simulink model "substation_132_13_8kv_digital_twin"  (R2023b)
settings: Solver=ode23tb  StartTime=0.0  StopTime=1.0  MaxStep=100e-6  RelTol=1e-3
settings Model: Creator=ASUS  LastModifiedBy=ASUS

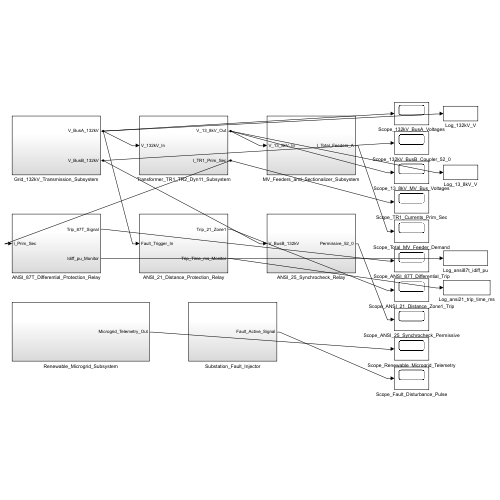
[thumbnail: Simulink's stored preview of the top-level diagram]
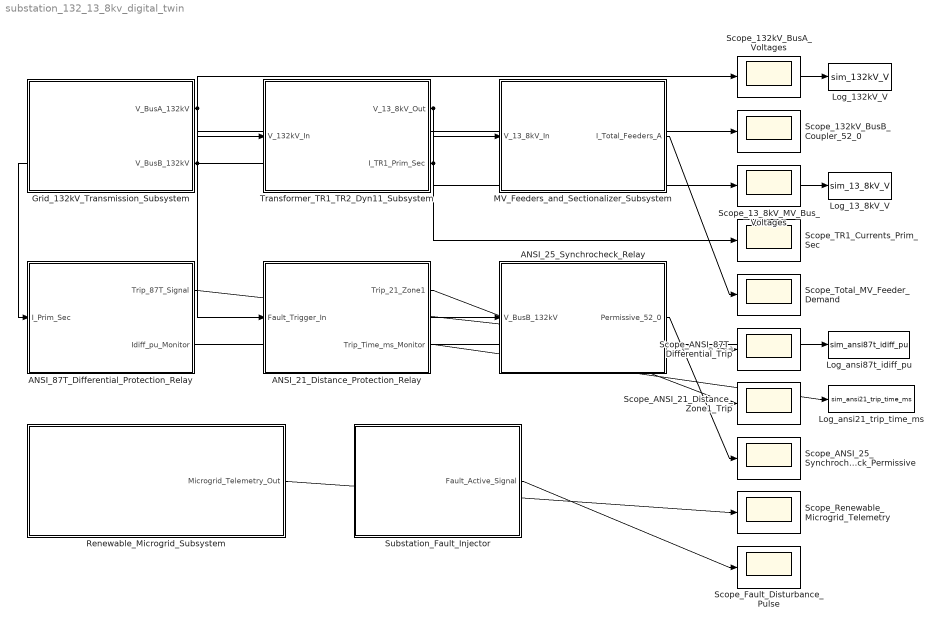
== system substation_132_13_8kv_digital_twin ==
  ANSI_21_Distance_Protection_Relay : Subsystem
  ANSI_25_Synchrocheck_Relay : Subsystem
  ANSI_87T_Differential_Protection_Relay : Subsystem
  Grid_132kV_Transmission_Subsystem : Subsystem
  Log_132kV_V : ToWorkspace  VariableName=sim_132kV_V  SampleTime=-1
  Log_13_8kV_V : ToWorkspace  VariableName=sim_13_8kV_V  SampleTime=-1
  Log_ansi21_trip_time_ms : ToWorkspace  VariableName=sim_ansi21_trip_time_ms  SampleTime=-1
  Log_ansi87t_idiff_pu : ToWorkspace  VariableName=sim_ansi87t_idiff_pu  SampleTime=-1
  MV_Feeders_and_Sectionalizer_Subsystem : Subsystem
  Renewable_Microgrid_Subsystem : Subsystem
  Scope_132kV_BusA_Voltages : Scope
  Scope_132kV_BusB_Coupler_52_0 : Scope
  Scope_13_8kV_MV_Bus_Voltages : Scope
  Scope_ANSI_21_Distance_Zone1_Trip : Scope
  Scope_ANSI_25_Synchrocheck_Permissive : Scope
  Scope_ANSI_87T_Differential_Trip : Scope
  Scope_Fault_Disturbance_Pulse : Scope
  Scope_Renewable_Microgrid_Telemetry : Scope
  Scope_TR1_Currents_Prim_Sec : Scope
  Scope_Total_MV_Feeder_Demand : Scope
  Substation_Fault_Injector : Subsystem
  Transformer_TR1_TR2_Dyn11_Subsystem : Subsystem
  wires:
  Grid_132kV_Transmission_Subsystem/1(V_BusA_132kV) -> Scope_132kV_BusA_Voltages/1, Log_132kV_V/1, Transformer_TR1_TR2_Dyn11_Subsystem/1(V_132kV_In), ANSI_21_Distance_Protection_Relay/1(Fault_Trigger_In)
  Grid_132kV_Transmission_Subsystem/2(V_BusB_132kV) -> Scope_132kV_BusB_Coupler_52_0/1, ANSI_25_Synchrocheck_Relay/1(V_BusB_132kV)
  Transformer_TR1_TR2_Dyn11_Subsystem/1(V_13_8kV_Out) -> Scope_13_8kV_MV_Bus_Voltages/1, Log_13_8kV_V/1, MV_Feeders_and_Sectionalizer_Subsystem/1(V_13_8kV_In)
  Transformer_TR1_TR2_Dyn11_Subsystem/2(I_TR1_Prim_Sec) -> Scope_TR1_Currents_Prim_Sec/1, ANSI_87T_Differential_Protection_Relay/1(I_Prim_Sec)
  MV_Feeders_and_Sectionalizer_Subsystem/1(I_Total_Feeders_A) -> Scope_Total_MV_Feeder_Demand/1
  ANSI_87T_Differential_Protection_Relay/1(Trip_87T_Signal) -> Scope_ANSI_87T_Differential_Trip/1
  ANSI_87T_Differential_Protection_Relay/2(Idiff_pu_Monitor) -> Log_ansi87t_idiff_pu/1
  ANSI_21_Distance_Protection_Relay/2(Trip_Time_ms_Monitor) -> Log_ansi21_trip_time_ms/1
  ANSI_21_Distance_Protection_Relay/1(Trip_21_Zone1) -> Scope_ANSI_21_Distance_Zone1_Trip/1
  ANSI_25_Synchrocheck_Relay/1(Permissive_52_0) -> Scope_ANSI_25_Synchrocheck_Permissive/1
  Renewable_Microgrid_Subsystem/1(Microgrid_Telemetry_Out) -> Scope_Renewable_Microgrid_Telemetry/1
  Substation_Fault_Injector/1(Fault_Active_Signal) -> Scope_Fault_Disturbance_Pulse/1

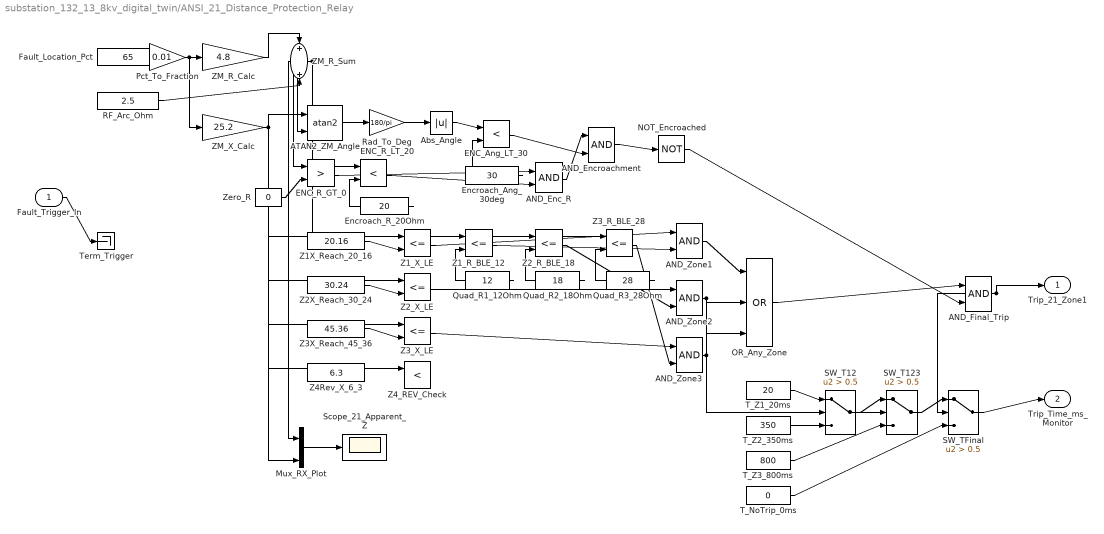
== system substation_132_13_8kv_digital_twin/ANSI_21_Distance_Protection_Relay ==
  Fault_Trigger_In : Inport
  AND_Enc_R : Logic  AllPortsSameDT=off  OutDataTypeStr=boolean
  AND_Encroachment : Logic  AllPortsSameDT=off  OutDataTypeStr=boolean
  AND_Final_Trip : Logic  AllPortsSameDT=off  OutDataTypeStr=boolean
  AND_Zone1 : Logic  AllPortsSameDT=off  OutDataTypeStr=boolean
  AND_Zone2 : Logic  AllPortsSameDT=off  OutDataTypeStr=boolean
  AND_Zone3 : Logic  AllPortsSameDT=off  OutDataTypeStr=boolean
  ATAN2_ZM_Angle : Trigonometry  Operator=atan2
  Abs_Angle : Abs  SaturateOnIntegerOverflow=off
  ENC_Ang_LT_30 : RelationalOperator  Operator=<  OutDataTypeStr=boolean  RndMeth=Simplest  InputSameDT=off
  ENC_R_GT_0 : RelationalOperator  Operator=>  OutDataTypeStr=boolean  RndMeth=Simplest  InputSameDT=off
  ENC_R_LT_20 : RelationalOperator  Operator=<  OutDataTypeStr=boolean  RndMeth=Simplest  InputSameDT=off
  Encroach_Ang_30deg : Constant  Value=30
  Encroach_R_20Ohm : Constant  Value=20
  Fault_Location_Pct : Constant  Value=65
  Mux_RX_Plot : Mux  Inputs=2
  NOT_Encroached : Logic  Operator=NOT  AllPortsSameDT=off  OutDataTypeStr=boolean
  OR_Any_Zone : Logic  Operator=OR  Inputs=3  AllPortsSameDT=off  OutDataTypeStr=boolean
  Pct_To_Fraction : Gain  Gain=0.01
  Quad_R1_12Ohm : Constant  Value=12
  Quad_R2_18Ohm : Constant  Value=18
  Quad_R3_28Ohm : Constant  Value=28
  RF_Arc_Ohm : Constant  Value=2.5
  Rad_To_Deg : Gain  Gain=180/pi
  SW_T12 : Switch  Criteria=u2 > Threshold  Threshold=0.5  SaturateOnIntegerOverflow=off  InputSameDT=off
  SW_T123 : Switch  Criteria=u2 > Threshold  Threshold=0.5  SaturateOnIntegerOverflow=off  InputSameDT=off
  SW_TFinal : Switch  Criteria=u2 > Threshold  Threshold=0.5  SaturateOnIntegerOverflow=off  InputSameDT=off
  Scope_21_Apparent_Z : Scope
  T_NoTrip_0ms : Constant  Value=0
  T_Z1_20ms : Constant  Value=20
  T_Z2_350ms : Constant  Value=350
  T_Z3_800ms : Constant  Value=800
  Term_Trigger : Terminator
  Z1X_Reach_20_16 : Constant  Value=20.16
  Z1_R_BLE_12 : RelationalOperator  Operator=<=  OutDataTypeStr=boolean  RndMeth=Simplest  InputSameDT=off
  Z1_X_LE : RelationalOperator  Operator=<=  OutDataTypeStr=boolean  RndMeth=Simplest  InputSameDT=off
  Z2X_Reach_30_24 : Constant  Value=30.24
  Z2_R_BLE_18 : RelationalOperator  Operator=<=  OutDataTypeStr=boolean  RndMeth=Simplest  InputSameDT=off
  Z2_X_LE : RelationalOperator  Operator=<=  OutDataTypeStr=boolean  RndMeth=Simplest  InputSameDT=off
  Z3X_Reach_45_36 : Constant  Value=45.36
  Z3_R_BLE_28 : RelationalOperator  Operator=<=  OutDataTypeStr=boolean  RndMeth=Simplest  InputSameDT=off
  Z3_X_LE : RelationalOperator  Operator=<=  OutDataTypeStr=boolean  RndMeth=Simplest  InputSameDT=off
  Z4Rev_X_6_3 : Constant  Value=6.3
  Z4_REV_Check : RelationalOperator  Operator=<  OutDataTypeStr=boolean  RndMeth=Simplest  InputSameDT=off
  ZM_R_Calc : Gain  Gain=4.8
  ZM_R_Sum : Sum
  ZM_X_Calc : Gain  Gain=25.2
  Zero_R : Constant  Value=0
  Trip_21_Zone1 : Outport
  Trip_Time_ms_Monitor : Outport  Port=2
  wires:
  Fault_Trigger_In/1 -> Term_Trigger/1
  Fault_Location_Pct/1 -> Pct_To_Fraction/1
  Pct_To_Fraction/1 -> ZM_R_Calc/1, ZM_X_Calc/1
  ZM_R_Calc/1 -> ZM_R_Sum/1
  RF_Arc_Ohm/1 -> ZM_R_Sum/2
  ZM_X_Calc/1 -> ATAN2_ZM_Angle/1, Z1_X_LE/1, Z2_X_LE/1, Z3_X_LE/1, Z4_REV_Check/1, Mux_RX_Plot/2
  ZM_R_Sum/1 -> ATAN2_ZM_Angle/2, ENC_R_GT_0/1, ENC_R_LT_20/1, Z1_R_BLE_12/1, Z2_R_BLE_18/1, Z3_R_BLE_28/1, Mux_RX_Plot/1
  ATAN2_ZM_Angle/1 -> Rad_To_Deg/1
  Rad_To_Deg/1 -> Abs_Angle/1
  Zero_R/1 -> ENC_R_GT_0/2
  Encroach_R_20Ohm/1 -> ENC_R_LT_20/2
  Abs_Angle/1 -> ENC_Ang_LT_30/1
  Encroach_Ang_30deg/1 -> ENC_Ang_LT_30/2
  ENC_R_GT_0/1 -> AND_Enc_R/1
  ENC_R_LT_20/1 -> AND_Enc_R/2
  AND_Enc_R/1 -> AND_Encroachment/1
  ENC_Ang_LT_30/1 -> AND_Encroachment/2
  Z1X_Reach_20_16/1 -> Z1_X_LE/2
  Z2X_Reach_30_24/1 -> Z2_X_LE/2
  Z3X_Reach_45_36/1 -> Z3_X_LE/2
  Quad_R1_12Ohm/1 -> Z1_R_BLE_12/2
  Quad_R2_18Ohm/1 -> Z2_R_BLE_18/2
  Quad_R3_28Ohm/1 -> Z3_R_BLE_28/2
  Z1_X_LE/1 -> AND_Zone1/1
  Z1_R_BLE_12/1 -> AND_Zone1/2
  Z2_X_LE/1 -> AND_Zone2/1
  Z2_R_BLE_18/1 -> AND_Zone2/2
  Z3_X_LE/1 -> AND_Zone3/1
  Z3_R_BLE_28/1 -> AND_Zone3/2
  AND_Zone1/1 -> OR_Any_Zone/1
  AND_Zone2/1 -> OR_Any_Zone/2, SW_T12/2
  AND_Zone3/1 -> OR_Any_Zone/3, SW_T123/2
  T_Z1_20ms/1 -> SW_T12/1
  T_Z2_350ms/1 -> SW_T12/3
  SW_T12/1 -> SW_T123/1
  T_Z3_800ms/1 -> SW_T123/3
  SW_T123/1 -> SW_TFinal/1
  AND_Final_Trip/1 -> SW_TFinal/2, Trip_21_Zone1/1
  T_NoTrip_0ms/1 -> SW_TFinal/3
  AND_Encroachment/1 -> NOT_Encroached/1
  OR_Any_Zone/1 -> AND_Final_Trip/1
  NOT_Encroached/1 -> AND_Final_Trip/2
  SW_TFinal/1 -> Trip_Time_ms_Monitor/1
  Mux_RX_Plot/1 -> Scope_21_Apparent_Z/1

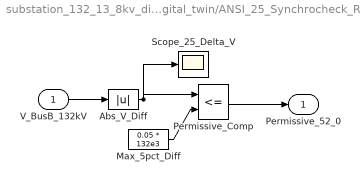
== system substation_132_13_8kv_digital_twin/ANSI_25_Synchrocheck_Relay ==
  V_BusB_132kV : Inport
  Abs_V_Diff : Abs  SaturateOnIntegerOverflow=off
  Max_5pct_Diff : Constant  Value=0.05 * 132e3
  Permissive_Comp : RelationalOperator  Operator=<=  OutDataTypeStr=boolean  RndMeth=Simplest  InputSameDT=off
  Scope_25_Delta_V : Scope
  Permissive_52_0 : Outport
  wires:
  Abs_V_Diff/1 -> Scope_25_Delta_V/1, Permissive_Comp/1
  V_BusB_132kV/1 -> Abs_V_Diff/1
  Max_5pct_Diff/1 -> Permissive_Comp/2
  Permissive_Comp/1 -> Permissive_52_0/1

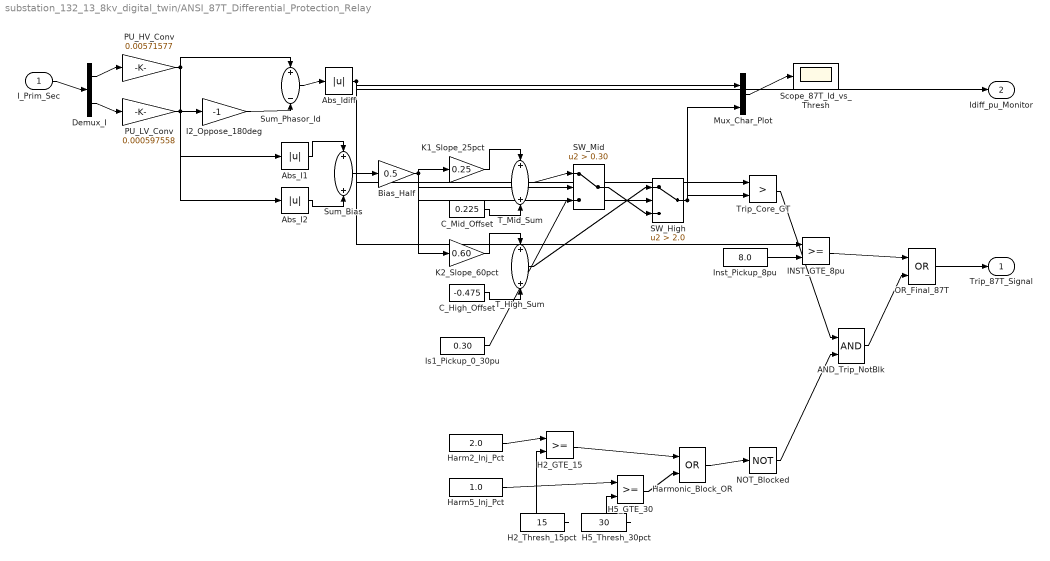
== system substation_132_13_8kv_digital_twin/ANSI_87T_Differential_Protection_Relay ==
  I_Prim_Sec : Inport
  AND_Trip_NotBlk : Logic  AllPortsSameDT=off  OutDataTypeStr=boolean
  Abs_I1 : Abs  SaturateOnIntegerOverflow=off
  Abs_I2 : Abs  SaturateOnIntegerOverflow=off
  Abs_Idiff : Abs  SaturateOnIntegerOverflow=off
  Bias_Half : Gain  Gain=0.5
  C_High_Offset : Constant  Value=-0.475
  C_Mid_Offset : Constant  Value=0.225
  Demux_I : Demux  Outputs=2
  H2_GTE_15 : RelationalOperator  OutDataTypeStr=boolean  RndMeth=Simplest  InputSameDT=off
  H2_Thresh_15pct : Constant  Value=15
  H5_GTE_30 : RelationalOperator  OutDataTypeStr=boolean  RndMeth=Simplest  InputSameDT=off
  H5_Thresh_30pct : Constant  Value=30
  Harm2_Inj_Pct : Constant  Value=2.0
  Harm5_Inj_Pct : Constant  Value=1.0
  Harmonic_Block_OR : Logic  Operator=OR  AllPortsSameDT=off  OutDataTypeStr=boolean
  I2_Oppose_180deg : Gain  Gain=-1
  INST_GTE_8pu : RelationalOperator  OutDataTypeStr=boolean  RndMeth=Simplest  InputSameDT=off
  Inst_Pickup_8pu : Constant  Value=8.0
  Is1_Pickup_0_30pu : Constant  Value=0.30
  K1_Slope_25pct : Gain  Gain=0.25
  K2_Slope_60pct : Gain  Gain=0.60
  Mux_Char_Plot : Mux  Inputs=2
  NOT_Blocked : Logic  Operator=NOT  AllPortsSameDT=off  OutDataTypeStr=boolean
  OR_Final_87T : Logic  Operator=OR  AllPortsSameDT=off  OutDataTypeStr=boolean
  PU_HV_Conv : Gain  Gain=0.00571577
  PU_LV_Conv : Gain  Gain=0.000597558
  SW_High : Switch  Criteria=u2 > Threshold  Threshold=2.0  SaturateOnIntegerOverflow=off  InputSameDT=off
  SW_Mid : Switch  Criteria=u2 > Threshold  Threshold=0.30  SaturateOnIntegerOverflow=off  InputSameDT=off
  Scope_87T_Id_vs_Thresh : Scope
  Sum_Bias : Sum
  Sum_Phasor_Id : Sum  Inputs=+-
  T_High_Sum : Sum
  T_Mid_Sum : Sum
  Trip_Core_GT : RelationalOperator  Operator=>  OutDataTypeStr=boolean  RndMeth=Simplest  InputSameDT=off
  Trip_87T_Signal : Outport
  Idiff_pu_Monitor : Outport  Port=2
  wires:
  I_Prim_Sec/1 -> Demux_I/1
  Demux_I/1 -> PU_HV_Conv/1
  Demux_I/2 -> PU_LV_Conv/1
  PU_LV_Conv/1 -> I2_Oppose_180deg/1, Abs_I2/1
  PU_HV_Conv/1 -> Sum_Phasor_Id/1, Abs_I1/1
  I2_Oppose_180deg/1 -> Sum_Phasor_Id/2
  Sum_Phasor_Id/1 -> Abs_Idiff/1
  Abs_I1/1 -> Sum_Bias/1
  Abs_I2/1 -> Sum_Bias/2
  Sum_Bias/1 -> Bias_Half/1
  Bias_Half/1 -> K1_Slope_25pct/1, K2_Slope_60pct/1, SW_Mid/2, SW_High/2
  K1_Slope_25pct/1 -> T_Mid_Sum/1
  C_Mid_Offset/1 -> T_Mid_Sum/2
  K2_Slope_60pct/1 -> T_High_Sum/1
  C_High_Offset/1 -> T_High_Sum/2
  T_Mid_Sum/1 -> SW_Mid/1
  Is1_Pickup_0_30pu/1 -> SW_Mid/3
  T_High_Sum/1 -> SW_High/1
  SW_Mid/1 -> SW_High/3
  Harm2_Inj_Pct/1 -> H2_GTE_15/1
  H2_Thresh_15pct/1 -> H2_GTE_15/2
  Harm5_Inj_Pct/1 -> H5_GTE_30/1
  H5_Thresh_30pct/1 -> H5_GTE_30/2
  H2_GTE_15/1 -> Harmonic_Block_OR/1
  H5_GTE_30/1 -> Harmonic_Block_OR/2
  Abs_Idiff/1 -> Trip_Core_GT/1, INST_GTE_8pu/1, Mux_Char_Plot/1, Idiff_pu_Monitor/1
  SW_High/1 -> Trip_Core_GT/2, Mux_Char_Plot/2
  Inst_Pickup_8pu/1 -> INST_GTE_8pu/2
  Harmonic_Block_OR/1 -> NOT_Blocked/1
  Trip_Core_GT/1 -> AND_Trip_NotBlk/1
  NOT_Blocked/1 -> AND_Trip_NotBlk/2
  INST_GTE_8pu/1 -> OR_Final_87T/1
  AND_Trip_NotBlk/1 -> OR_Final_87T/2
  OR_Final_87T/1 -> Trip_87T_Signal/1
  Mux_Char_Plot/1 -> Scope_87T_Id_vs_Thresh/1

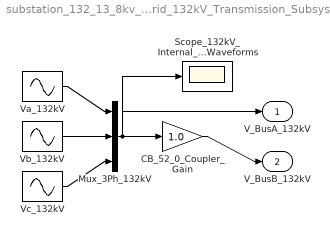
== system substation_132_13_8kv_digital_twin/Grid_132kV_Transmission_Subsystem ==
  CB_52_0_Coupler_Gain : Gain  Gain=1.0
  Mux_3Ph_132kV : Mux  Inputs=3
  Scope_132kV_Internal_Waveforms : Scope
  Va_132kV : Sin  Amplitude=132e3 * sqrt(2)/sqrt(3)  Frequency=2*pi*60  SampleTime=0
  Vb_132kV : Sin  Amplitude=132e3 * sqrt(2)/sqrt(3)  Frequency=2*pi*60  Phase=-2*pi/3  SampleTime=0
  Vc_132kV : Sin  Amplitude=132e3 * sqrt(2)/sqrt(3)  Frequency=2*pi*60  Phase=2*pi/3  SampleTime=0
  V_BusA_132kV : Outport
  V_BusB_132kV : Outport  Port=2
  wires:
  Mux_3Ph_132kV/1 -> Scope_132kV_Internal_Waveforms/1, V_BusA_132kV/1, CB_52_0_Coupler_Gain/1
  Va_132kV/1 -> Mux_3Ph_132kV/1
  Vb_132kV/1 -> Mux_3Ph_132kV/2
  Vc_132kV/1 -> Mux_3Ph_132kV/3
  CB_52_0_Coupler_Gain/1 -> V_BusB_132kV/1

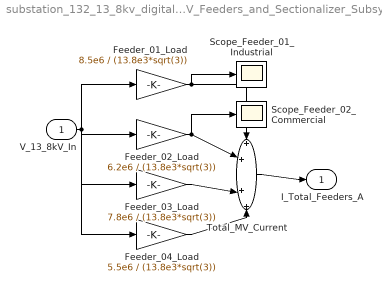
== system substation_132_13_8kv_digital_twin/MV_Feeders_and_Sectionalizer_Subsystem ==
  V_13_8kV_In : Inport
  Feeder_01_Load : Gain  Gain=8.5e6 / (13.8e3*sqrt(3))
  Feeder_02_Load : Gain  Gain=6.2e6 / (13.8e3*sqrt(3))
  Feeder_03_Load : Gain  Gain=7.8e6 / (13.8e3*sqrt(3))
  Feeder_04_Load : Gain  Gain=5.5e6 / (13.8e3*sqrt(3))
  Scope_Feeder_01_Industrial : Scope
  Scope_Feeder_02_Commercial : Scope
  Total_MV_Current : Sum  Inputs=++++
  I_Total_Feeders_A : Outport
  wires:
  Feeder_01_Load/1 -> Scope_Feeder_01_Industrial/1, Total_MV_Current/1
  Feeder_02_Load/1 -> Scope_Feeder_02_Commercial/1, Total_MV_Current/2
  V_13_8kV_In/1 -> Feeder_01_Load/1, Feeder_02_Load/1, Feeder_03_Load/1, Feeder_04_Load/1
  Feeder_03_Load/1 -> Total_MV_Current/3
  Feeder_04_Load/1 -> Total_MV_Current/4
  Total_MV_Current/1 -> I_Total_Feeders_A/1

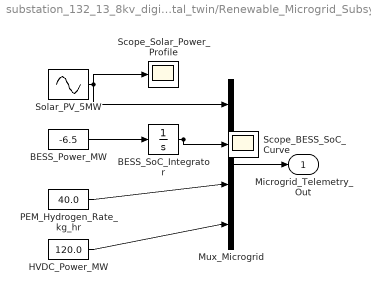
== system substation_132_13_8kv_digital_twin/Renewable_Microgrid_Subsystem ==
  BESS_Power_MW : Constant  Value=-6.5
  BESS_SoC_Integrator : Integrator  InitialCondition=72.0
  HVDC_Power_MW : Constant  Value=120.0
  Mux_Microgrid : Mux
  PEM_Hydrogen_Rate_kg_hr : Constant  Value=40.0
  Scope_BESS_SoC_Curve : Scope
  Scope_Solar_Power_Profile : Scope
  Solar_PV_5MW : Sin  Amplitude=5.0  Frequency=2*pi/24  Phase=-pi/2  SampleTime=0
  Microgrid_Telemetry_Out : Outport
  wires:
  Solar_PV_5MW/1 -> Scope_Solar_Power_Profile/1, Mux_Microgrid/1
  BESS_SoC_Integrator/1 -> Scope_BESS_SoC_Curve/1, Mux_Microgrid/2
  BESS_Power_MW/1 -> BESS_SoC_Integrator/1
  PEM_Hydrogen_Rate_kg_hr/1 -> Mux_Microgrid/3
  HVDC_Power_MW/1 -> Mux_Microgrid/4
  Mux_Microgrid/1 -> Microgrid_Telemetry_Out/1

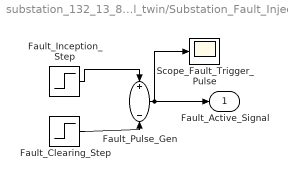
== system substation_132_13_8kv_digital_twin/Substation_Fault_Injector ==
  Fault_Clearing_Step : Step  Time=0.28  SampleTime=0
  Fault_Inception_Step : Step  Time=0.20  SampleTime=0
  Fault_Pulse_Gen : Sum  Inputs=+-
  Scope_Fault_Trigger_Pulse : Scope
  Fault_Active_Signal : Outport
  wires:
  Fault_Pulse_Gen/1 -> Scope_Fault_Trigger_Pulse/1, Fault_Active_Signal/1
  Fault_Inception_Step/1 -> Fault_Pulse_Gen/1
  Fault_Clearing_Step/1 -> Fault_Pulse_Gen/2

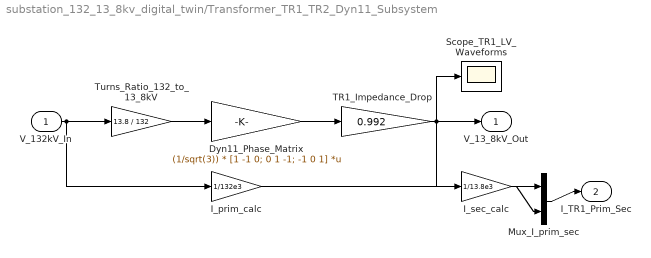
== system substation_132_13_8kv_digital_twin/Transformer_TR1_TR2_Dyn11_Subsystem ==
  V_132kV_In : Inport
  Dyn11_Phase_Matrix : Gain  Gain=(1/sqrt(3)) * [1 -1 0; 0 1 -1; -1 0 1]  Multiplication=Matrix(K*u)
  I_prim_calc : Gain  Gain=1/132e3
  I_sec_calc : Gain  Gain=1/13.8e3
  Mux_I_prim_sec : Mux  Inputs=2
  Scope_TR1_LV_Waveforms : Scope
  TR1_Impedance_Drop : Gain  Gain=0.992
  Turns_Ratio_132_to_13_8kV : Gain  Gain=13.8 / 132
  V_13_8kV_Out : Outport
  I_TR1_Prim_Sec : Outport  Port=2
  wires:
  TR1_Impedance_Drop/1 -> Scope_TR1_LV_Waveforms/1, V_13_8kV_Out/1, I_sec_calc/1
  V_132kV_In/1 -> Turns_Ratio_132_to_13_8kV/1, I_prim_calc/1
  Turns_Ratio_132_to_13_8kV/1 -> Dyn11_Phase_Matrix/1
  Dyn11_Phase_Matrix/1 -> TR1_Impedance_Drop/1
  I_prim_calc/1 -> Mux_I_prim_sec/1
  I_sec_calc/1 -> Mux_I_prim_sec/2
  Mux_I_prim_sec/1 -> I_TR1_Prim_Sec/1
